simulink model "FULL_SIMULATION"  (R2025b)
settings: Solver=VariableStepAuto  StartTime=0.0  StopTime=10.0  RelTol=1e-3
InitFcn:
  | p_init  = [0,0,0];
  | v_init  = [0,0,0];
  | q_init  = [1,0,0,0];
  | bg_init = [1.045715,0.002947,-0.517855];
  | ba_high_init = [-7.395250,-4.820243,-18.177021];
  | ba_low_init = [-0.021725, 0.062643, -0.022747];
  | 
  | taug_init = [1.105; 1.105; 1.105];
  | taua_high_init = [8.731; 8.731; 8.731];
  | taua_low_init = [1.437; 1.437; 1.437];
  | qg_init = [4.390573e-05; 2.319960e-05; 1.494807e-05];
  | qa_high_init = [8.774166e-04; 7.720775e-04; 1.336849e-03];
  | qa_low_init = [1.483796e-06; 1.224280e-06; 1.983171e-06];
  | 
  | 
  | x_init = [p_init, v_init, q_init, bg_init, ba_high_init, ba_low_init]';
  | P_init = zeros(19);
  | dt = 1 / 120;
libraries: aerolibutil x1
settings Model: Creator=Admin  LastModifiedBy=Admin

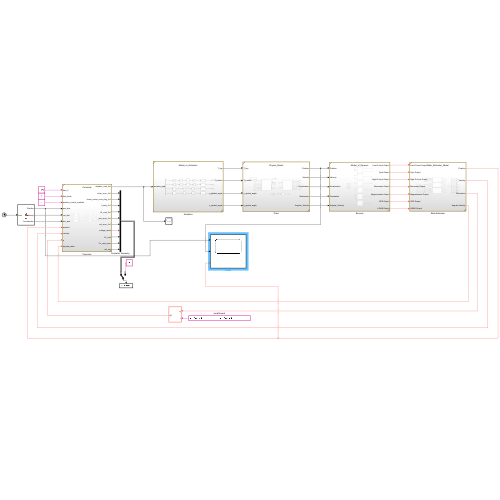
[thumbnail: Simulink's stored preview of the top-level diagram]
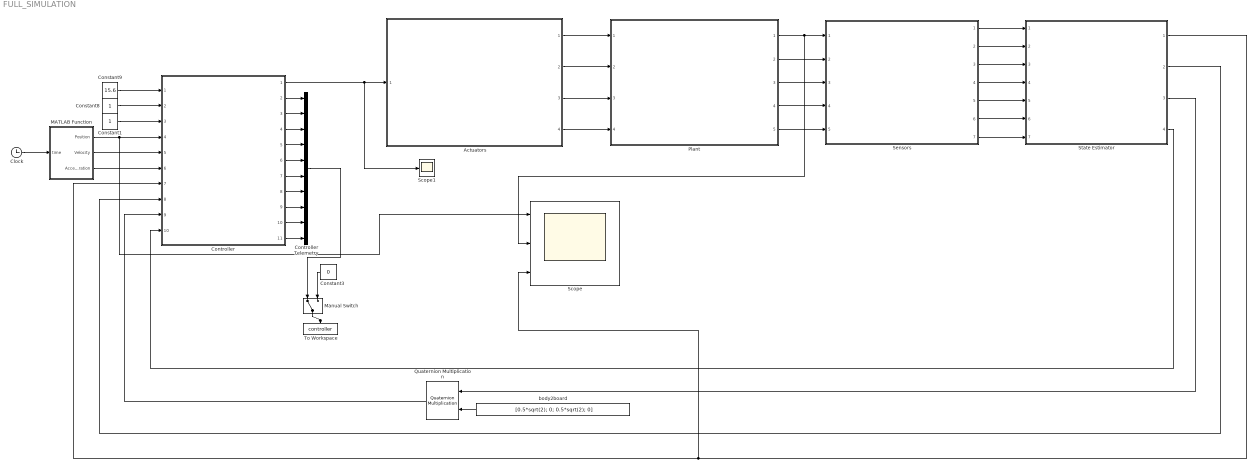
== system FULL_SIMULATION ==
  Actuators : Subsystem  ReferencedSubsystem=Model_of_Actuators
  Clock : Clock
  Constant1 : Constant
  Constant3 : Constant  Value=0
  Constant8 : Constant
  Constant9 : Constant  Value=15.6
  Controller : Subsystem  ReferencedSubsystem=Controller
  Controller Telemetry : BusCreator  Inputs=10
  MATLAB Function : MATLAB Function  TreatAsAtomicUnit=on
  Manual Switch : ManualSwitch
  Plant : Subsystem  ReferencedSubsystem=Physics_Model
  Quaternion Multiplication : aerolibutil/Quaternion Multiplication
  Scope : Scope  NumInputPorts=3
      settings: ActiveDisplayYMinimum=-121.34051499924058  ActiveDisplayYMaximum=176.92909024017214
  Scope1 : Scope
      settings: ActiveDisplayYMinimum=-1  ActiveDisplayYMaximum=1
  Sensors : Subsystem  ReferencedSubsystem=Model_of_Sensors
  State Estimator : Subsystem  ReferencedSubsystem=State_Estimator_Model
  To Workspace : ToWorkspace  VariableName=controller  SaveFormat=Timeseries  SampleTime=-1
  body2board : Constant  Value=[0.5*sqrt(2); 0; 0.5*sqrt(2); 0]
  wires:
  Plant/1 -> Scope/2, Sensors/1
  Plant/2 -> Sensors/2
  Plant/3 -> Sensors/3
  Plant/4 -> Sensors/4
  Plant/5 -> Sensors/5
  Sensors/1 -> State Estimator/1
  Sensors/2 -> State Estimator/2
  Sensors/3 -> State Estimator/3
  Sensors/4 -> State Estimator/4
  Sensors/5 -> State Estimator/5
  Sensors/6 -> State Estimator/6
  Sensors/7 -> State Estimator/7
  Controller/2 -> Controller Telemetry/1
  Controller/3 -> Controller Telemetry/2
  Controller/4 -> Controller Telemetry/3
  Controller/5 -> Controller Telemetry/4
  Controller/6 -> Controller Telemetry/5
  Controller/7 -> Controller Telemetry/6
  Controller/8 -> Controller Telemetry/7
  Controller/9 -> Controller Telemetry/8
  Controller/10 -> Controller Telemetry/9
  Controller/11 -> Controller Telemetry/10
  Controller Telemetry/1 -> Manual Switch/1
  Manual Switch/1 -> To Workspace/1
  Constant3/1 -> Manual Switch/2
  body2board/1 -> Quaternion Multiplication/2
  Quaternion Multiplication/1 -> Controller/9
  Controller/1 -> Scope1/1, Actuators/1
  Actuators/1 -> Plant/1
  Actuators/2 -> Plant/2
  Actuators/3 -> Plant/3
  Actuators/4 -> Plant/4
  State Estimator/3 -> Quaternion Multiplication/1
  State Estimator/1 -> Scope/3, Controller/7
  State Estimator/2 -> Controller/8
  State Estimator/4 -> Controller/10
  Constant8/1 -> Controller/2
  Constant9/1 -> Controller/1
  Constant1/1 -> Controller/3
  MATLAB Function/3(Acceleration) -> Controller/6
  MATLAB Function/2(Velocity) -> Controller/5
  MATLAB Function/1(Position) -> Scope/1, Controller/4
  Clock/1 -> MATLAB Function/1(time)

== matlab function FULL_SIMULATION/MATLAB Function ==
  data: time input; Position output; Velocity output; Acceleration output
function [Position, Velocity, Acceleration] = fcn(time)
% Frames:
% - Position, Velocity, Acceleration in NED
% - Quaternion scalar-first [q0; q1; q2; q3]
% - Angular_Velocity = [p; q; r] in rad/s

% -----------------------------
% Trajectory configuration
% -----------------------------
T.x0       = 0.0;   T.xi = 2.0;   T.xf = 0.0;
T.y0       = 0.0;   T.yi = 2.0;   T.yf = 0.0;
T.z0       = 0.0;   T.zi = -2.0;   T.zf = 0.0;
T.t1       = 5.0;
T.t2       = 5.0;
T.dt_blend = 2.0;
T.frac_tb  = 0.20;
T.useStep  = false;

% -----------------------------
% Translational motion
% -----------------------------
[Position, Velocity, Acceleration] = trapezoidalRefBlockXYZ(time, T);
